simulink model "TP_manual_vrx"  (R2024b)
settings: Solver=FixedStepDiscrete  StartTime=0.0  StopTime=T_end_tp  FixedStep=Ts_tp  RelTol=1e-3
PostLoadFcn:
  | addpath(fileparts(get_param('TP_manual_vrx','FileName')));
InitFcn:
  | TP_manual_init('TP_manual_vrx');
StopFcn:
  | TP_manual_stop('TP_manual_vrx');
values from neighbouring files (symbols this model uses):
  alloc_prm = [half_beam; l_bow; F_max; F_bow_max]    [TP_manual_setup.m]
  D = G.D(1:G.n, :)    [TP_gcs.m]
  d_gps = 0.85    [TP_manual_setup.m]
  lat0_tp = 35.1862095    [TP_manual_setup.m]
  lon0_tp = 128.5665903    [TP_manual_setup.m]
  N_btn = 400    [TP_manual_setup.m]
  S = struct('n', 0)    [TP_gcs.m]    (also in TP_manual_check.m = TP_gcs('result'); TP_manual_stop.m = TP_gcs('result'); TP_mission.m = TP_gcs('result'))
  Ts_tp = 0.05    [TP_manual_setup.m]
  W = 1 - e2*sind(lat0)^2    [TP_gcs.m]    (also in TP_make_video.m = [])
  X_btn = 400    [TP_manual_setup.m]
  Y_btn = 200    [TP_manual_setup.m]
undefined symbols (not defined in the file or in its folder): A, Q
libraries: ros2lib x8
settings Model: Creator=wkyou  LastModifiedBy=wkyou

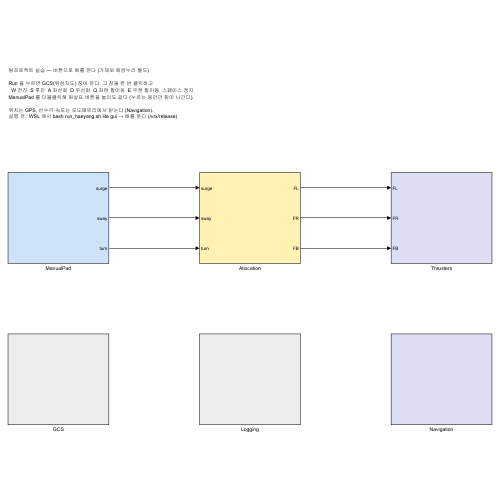
[thumbnail: Simulink's stored preview of the top-level diagram]
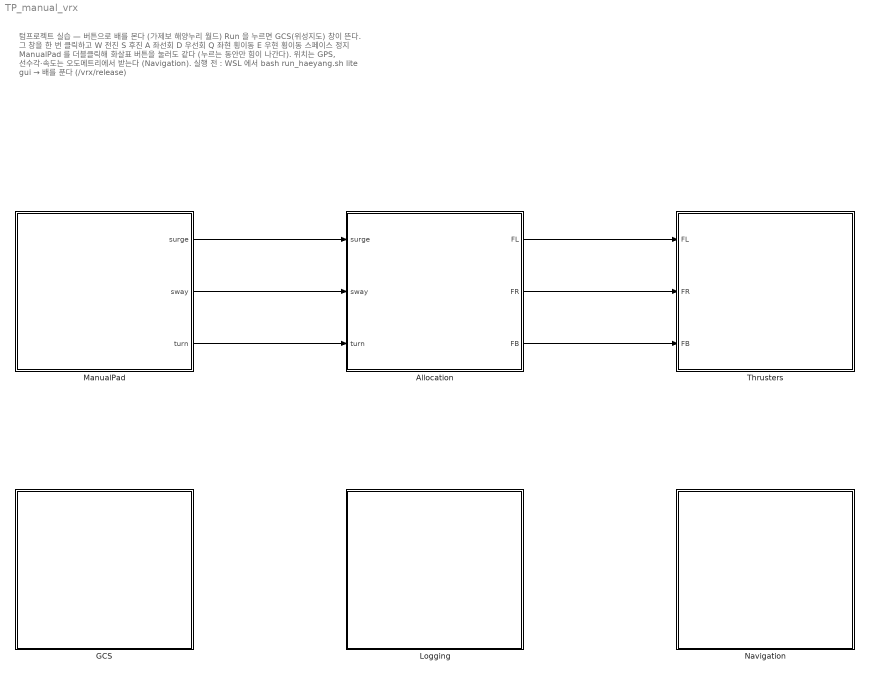
== system TP_manual_vrx ==
  note: 텀프로젝트 실습 — 버튼으로 배를 몬다 (가제보 해양누리 월드)
      |
      | Run 을 누르면 GCS(위성지도) 창이 뜬다. 그 창을 한 번 클릭하고
      |   W 전진  S 후진  A 좌선회  D 우선회  Q 좌현 횡이동  E 우현 횡이동  스페이스 정지
      | ManualPad 를 더블클릭해 화살표 버튼을 눌러도 같다 (누르는 동안만 힘이 나간다).
      |
      | 위치는 GPS, 선수각·속도는 오도메트리에서 받는다 (Navigation).
      | 실행 전 : WSL 에서 bash run_haeyang.sh lite gui → 배를 푼다 (/vrx/release)
  Allocation : Subsystem
  GCS : Subsystem
  Logging : Subsystem
  ManualPad : Subsystem
  Navigation : Subsystem
  Thrusters : Subsystem
  wires:
  ManualPad/1(surge) -> Allocation/1(surge)
  Allocation/1(FL) -> Thrusters/1(FL)
  ManualPad/2(sway) -> Allocation/2(sway)
  Allocation/2(FR) -> Thrusters/2(FR)
  ManualPad/3(turn) -> Allocation/3(turn)
  Allocation/3(FB) -> Thrusters/3(FB)

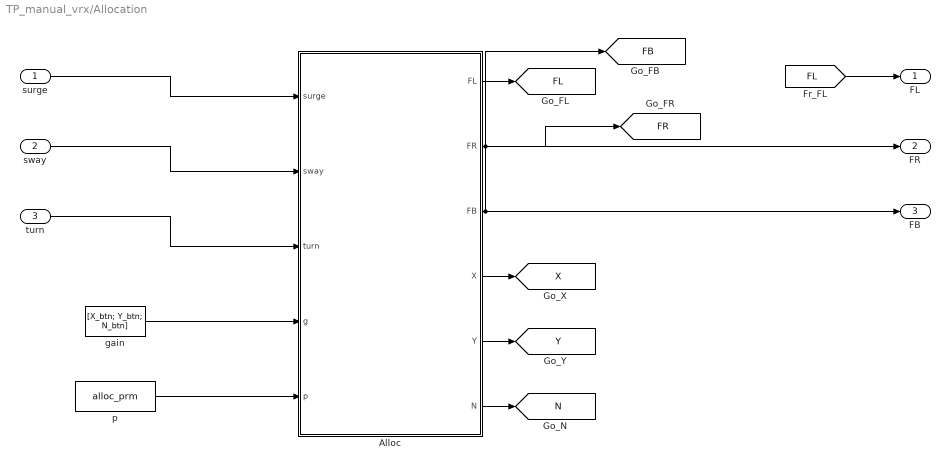
== system TP_manual_vrx/Allocation ==
  surge : Inport
  sway : Inport  Port=2
  turn : Inport  Port=3
  Alloc : MATLAB Function  TreatAsAtomicUnit=on
  gain : Constant  Value=[X_btn; Y_btn; N_btn]
  p : Constant  Value=alloc_prm
  FL : Outport
  FR : Outport  Port=2
  FB : Outport  Port=3
  tag scope: FB=global, FL=global, FR=global, N=global, X=global, Y=global
  wires:
  surge/1 -> Alloc/1(surge)
  sway/1 -> Alloc/2(sway)
  turn/1 -> Alloc/3(turn)
  gain/1 -> Alloc/4(g)
  p/1 -> Alloc/5(p)
  Alloc/2(FR) -> [FR], FR/1
  Alloc/3(FB) -> FB/1, [FB]
  Alloc/1(FL) -> [FL]
  Alloc/6(N) -> [N]
  Alloc/4(X) -> [X]
  Alloc/5(Y) -> [Y]
  [FL] -> FL/1

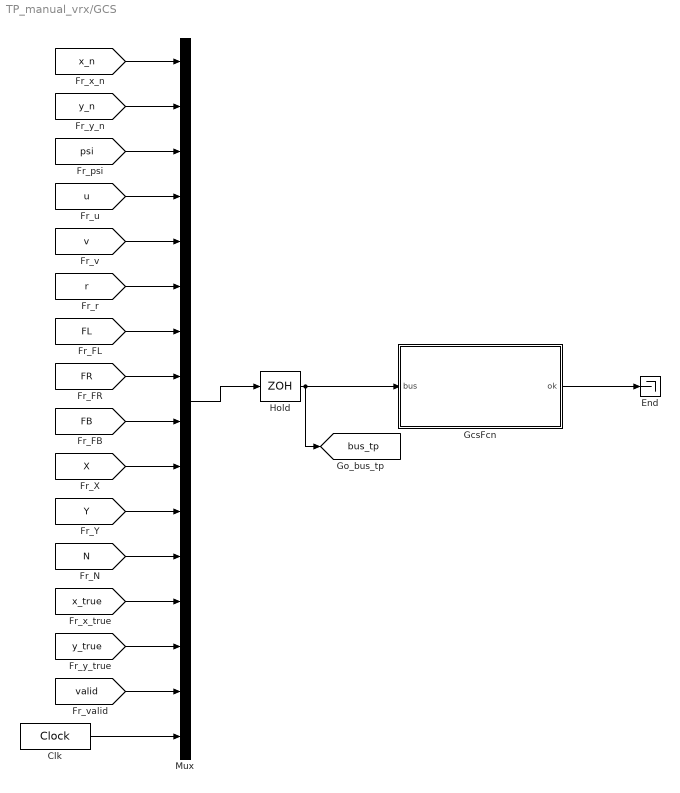
== system TP_manual_vrx/GCS ==
  Clk : DigitalClock  SampleTime=Ts_tp
  End : Terminator
  GcsFcn : MATLAB Function  TreatAsAtomicUnit=on
  Hold : ZeroOrderHold  SampleTime=Ts_tp
  Mux : Mux  Inputs=16
  tag scope: bus_tp=global
  wires:
  Clk/1 -> Mux/16
  Mux/1 -> Hold/1
  Hold/1 -> GcsFcn/1(bus), [bus_tp]
  GcsFcn/1(ok) -> End/1
  [FB] -> Mux/9
  [FL] -> Mux/7
  [FR] -> Mux/8
  [N] -> Mux/12
  [X] -> Mux/10
  [Y] -> Mux/11
  [psi] -> Mux/3
  [r] -> Mux/6
  [u] -> Mux/4
  [v] -> Mux/5
  [valid] -> Mux/15
  [x_n] -> Mux/1
  [x_true] -> Mux/13
  [y_n] -> Mux/2
  [y_true] -> Mux/14

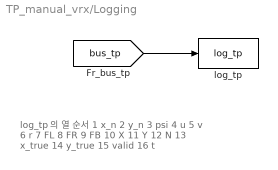
== system TP_manual_vrx/Logging ==
  note: log_tp 의 열 순서
      |  1 x_n   2 y_n   3 psi   4 u   5 v   6 r
      |  7 FL    8 FR    9 FB   10 X  11 Y  12 N
      | 13 x_true  14 y_true  15 valid  16 t
  log_tp : ToWorkspace  VariableName=log_tp  SaveFormat=Timeseries  SampleTime=Ts_tp
  wires:
  [bus_tp] -> log_tp/1

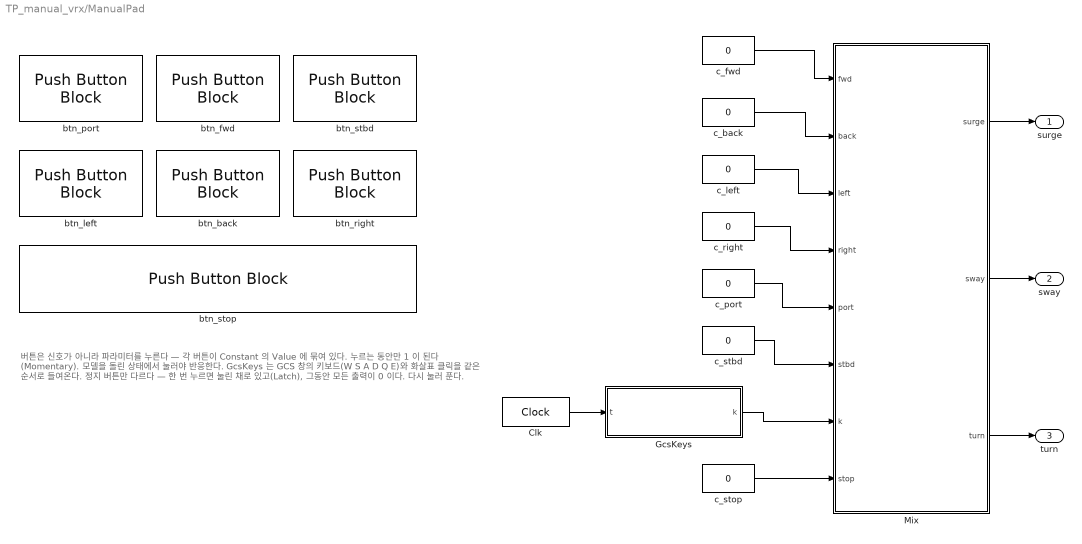
== system TP_manual_vrx/ManualPad ==
  note: 버튼은 신호가 아니라 파라미터를 누른다 — 각 버튼이 Constant 의 Value 에 묶여 있다.
      | 누르는 동안만 1 이 된다 (Momentary). 모델을 돌린 상태에서 눌러야 반응한다.
      | GcsKeys 는 GCS 창의 키보드(W S A D Q E)와 화살표 클릭을 같은 순서로 들여온다.
      | 정지 버튼만 다르다 — 한 번 누르면 눌린 채로 있고(Latch), 그동안 모든 출력이 0 이다. 다시 눌러 푼다.
  Clk : DigitalClock  SampleTime=Ts_tp
  GcsKeys : MATLAB Function  TreatAsAtomicUnit=on
  Mix : MATLAB Function  TreatAsAtomicUnit=on
  btn_back : PushButtonBlock  ButtonText=▼ 후진 (S)
  btn_fwd : PushButtonBlock  ButtonText=▲ 전진 (W)
  btn_left : PushButtonBlock  ButtonText=◀ 좌선회 (A)
  btn_port : PushButtonBlock  ButtonText=⇦ 좌현 횡 (Q)
  btn_right : PushButtonBlock  ButtonText=▶ 우선회 (D)
  btn_stbd : PushButtonBlock  ButtonText=⇨ 우현 횡 (E)
  btn_stop : PushButtonBlock  ButtonText="■ 정지 — 모든 출력 0  (다시 누르면 풀림)"  ButtonType=Latch
  c_back : Constant  Value=0
  c_fwd : Constant  Value=0
  c_left : Constant  Value=0
  c_port : Constant  Value=0
  c_right : Constant  Value=0
  c_stbd : Constant  Value=0
  c_stop : Constant  Value=0
  surge : Outport
  sway : Outport  Port=2
  turn : Outport  Port=3
  wires:
  c_back/1 -> Mix/2(back)
  Clk/1 -> GcsKeys/1(t)
  Mix/3(turn) -> turn/1
  c_fwd/1 -> Mix/1(fwd)
  c_port/1 -> Mix/5(port)
  c_left/1 -> Mix/3(left)
  c_right/1 -> Mix/4(right)
  c_stbd/1 -> Mix/6(stbd)
  c_stop/1 -> Mix/8(stop)
  GcsKeys/1(k) -> Mix/7(k)
  Mix/1(surge) -> surge/1
  Mix/2(sway) -> sway/1

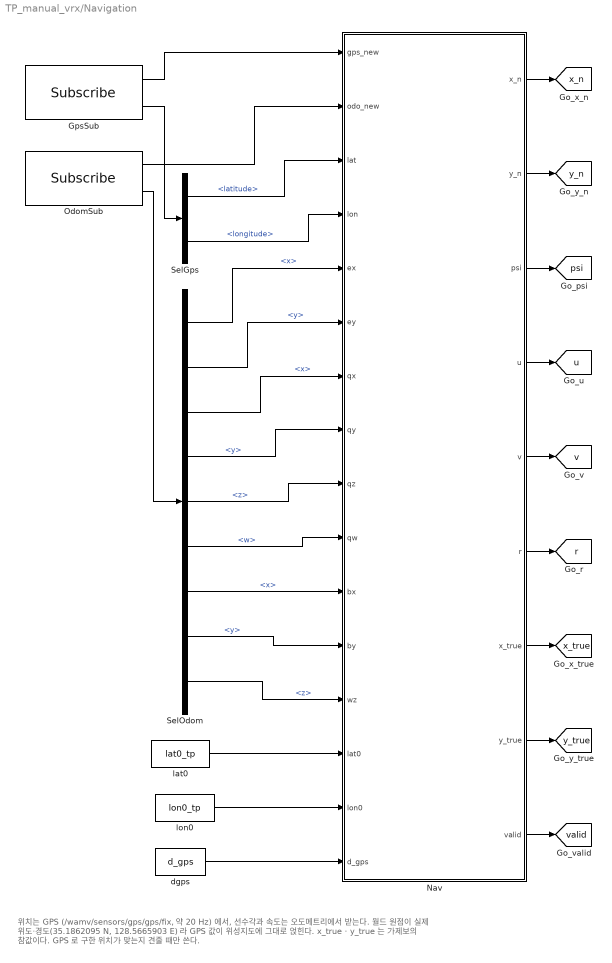
== system TP_manual_vrx/Navigation ==
  note: 위치는 GPS (/wamv/sensors/gps/gps/fix, 약 20 Hz) 에서, 선수각과 속도는 오도메트리에서 받는다.
      | 월드 원점이 실제 위도·경도(35.1862095 N, 128.5665903 E)라 GPS 값이 위성지도에 그대로 얹힌다.
      | x_true · y_true 는 가제보의 참값이다. GPS 로 구한 위치가 맞는지 견줄 때만 쓴다.
  GpsSub : ros2lib/Subscribe  topicSource=Specify your own  topic=/wamv/sensors/gps/gps/fix  messageType=sensor_msgs/NavSatFix  sampleTime=Ts_tp  QOSHistory=Keep last  QOSDepth=1  QOSReliability=Reliable  QOSDurability=Volatile  QOSDeadline=Inf  QOSLifespan=Inf  QOSLiveliness=Automatic  QOSLeaseDuration=Inf  QOSAvoidROSNamespaceConventions=off
  Nav : MATLAB Function  TreatAsAtomicUnit=on
  OdomSub : ros2lib/Subscribe  topicSource=Specify your own  topic=/wamv/sensors/position/ground_truth_odometry  messageType=nav_msgs/Odometry  sampleTime=Ts_tp  QOSHistory=Keep last  QOSDepth=1  QOSReliability=Reliable  QOSDurability=Volatile  QOSDeadline=Inf  QOSLifespan=Inf  QOSLiveliness=Automatic  QOSLeaseDuration=Inf  QOSAvoidROSNamespaceConventions=off
  SelGps : BusSelector  OutputSignals=latitude,longitude
  SelOdom : BusSelector  OutputSignals=pose.pose.position.x,pose.pose.position.y,pose.pose.orientation.x,pose.pose.orientation.y,pose.pose.orientation.z,pose.pose.orientation.w,twist.twist.linear.x,twist.twist.linear.y,twist.twist.angular.z
  dgps : Constant  Value=d_gps
  lat0 : Constant  Value=lat0_tp
  lon0 : Constant  Value=lon0_tp
  tag scope: psi=global, r=global, u=global, v=global, valid=global, x_n=global, x_true=global, y_n=global, y_true=global
  wires:
  OdomSub/2 -> SelOdom/1
  GpsSub/1 -> Nav/1(gps_new)
  SelGps/1 -> Nav/3(lat)  "<latitude>"
  SelOdom/2 -> Nav/6(ey)  "<y>"
  GpsSub/2 -> SelGps/1
  OdomSub/1 -> Nav/2(odo_new)
  SelGps/2 -> Nav/4(lon)  "<longitude>"
  SelOdom/9 -> Nav/13(wz)  "<z>"
  SelOdom/1 -> Nav/5(ex)  "<x>"
  SelOdom/3 -> Nav/7(qx)  "<x>"
  SelOdom/4 -> Nav/8(qy)  "<y>"
  SelOdom/5 -> Nav/9(qz)  "<z>"
  SelOdom/6 -> Nav/10(qw)  "<w>"
  SelOdom/7 -> Nav/11(bx)  "<x>"
  SelOdom/8 -> Nav/12(by)  "<y>"
  lat0/1 -> Nav/14(lat0)
  lon0/1 -> Nav/15(lon0)
  dgps/1 -> Nav/16(d_gps)
  Nav/3(psi) -> [psi]
  Nav/6(r) -> [r]
  Nav/4(u) -> [u]
  Nav/5(v) -> [v]
  Nav/9(valid) -> [valid]
  Nav/1(x_n) -> [x_n]
  Nav/7(x_true) -> [x_true]
  Nav/2(y_n) -> [y_n]
  Nav/8(y_true) -> [y_true]

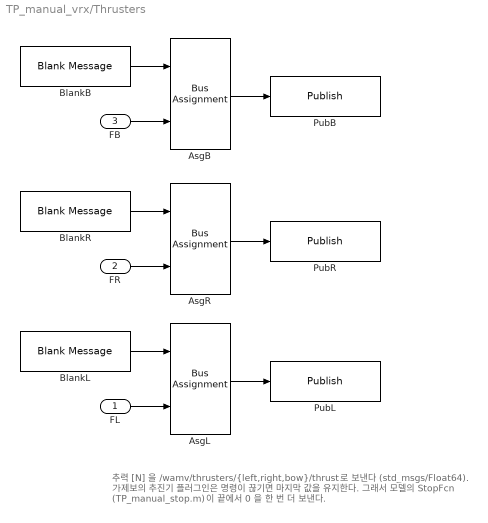
== system TP_manual_vrx/Thrusters ==
  note: 추력 [N] 을 /wamv/thrusters/{left,right,bow}/thrust 로 보낸다 (std_msgs/Float64).
      | 가제보의 추진기 플러그인은 명령이 끊기면 마지막 값을 유지한다.
      | 그래서 모델의 StopFcn (TP_manual_stop.m) 이 끝에서 0 을 한 번 더 보낸다.
  FL : Inport
  FR : Inport  Port=2
  FB : Inport  Port=3
  AsgB : BusAssignment  AssignedSignals=data
  AsgL : BusAssignment  AssignedSignals=data
  AsgR : BusAssignment  AssignedSignals=data
  BlankB : ros2lib/Blank Message  messageClass=Message  entityType=std_msgs/Float64  messageType=std_msgs/Float64  SampleTime=Ts_tp
  BlankL : ros2lib/Blank Message  messageClass=Message  entityType=std_msgs/Float64  messageType=std_msgs/Float64  SampleTime=Ts_tp
  BlankR : ros2lib/Blank Message  messageClass=Message  entityType=std_msgs/Float64  messageType=std_msgs/Float64  SampleTime=Ts_tp
  PubB : ros2lib/Publish  topicSource=Specify your own  topic=/wamv/thrusters/bow/thrust  messageType=std_msgs/Float64  QOSHistory=Keep last  QOSDepth=1  QOSReliability=Reliable  QOSDurability=Volatile  QOSDeadline=Inf  QOSLifespan=Inf  QOSLiveliness=Automatic  QOSLeaseDuration=Inf  QOSAvoidROSNamespaceConventions=off
  PubL : ros2lib/Publish  topicSource=Specify your own  topic=/wamv/thrusters/left/thrust  messageType=std_msgs/Float64  QOSHistory=Keep last  QOSDepth=1  QOSReliability=Reliable  QOSDurability=Volatile  QOSDeadline=Inf  QOSLifespan=Inf  QOSLiveliness=Automatic  QOSLeaseDuration=Inf  QOSAvoidROSNamespaceConventions=off
  PubR : ros2lib/Publish  topicSource=Specify your own  topic=/wamv/thrusters/right/thrust  messageType=std_msgs/Float64  QOSHistory=Keep last  QOSDepth=1  QOSReliability=Reliable  QOSDurability=Volatile  QOSDeadline=Inf  QOSLifespan=Inf  QOSLiveliness=Automatic  QOSLeaseDuration=Inf  QOSAvoidROSNamespaceConventions=off
  wires:
  BlankR/1 -> AsgR/1
  BlankB/1 -> AsgB/1
  FB/1 -> AsgB/2
  FR/1 -> AsgR/2
  BlankL/1 -> AsgL/1
  AsgR/1 -> PubR/1
  AsgB/1 -> PubB/1
  FL/1 -> AsgL/2
  AsgL/1 -> PubL/1

== matlab function TP_manual_vrx/ManualPad/Mix ==
  data: fwd input; surge output; back input; left input; right input; port input; stbd input; k input; stop input; sway output; turn output
function [surge, sway, turn] = Mix(fwd, back, left, right, port, stbd, k, stop)
%#codegen
% 버튼 여섯(이 상자의 Push Button)과 GCS 창의 입력 k 를 합친다.
% 어느 쪽에서 누르든 같다 — 하나라도 눌리면 1.
b = min(1, [fwd; back; left; right; port; stbd] + k);

surge = b(1) - b(2);     % 전진 +1, 후진 -1
sway  = b(6) - b(5);     % 우현 +1, 좌현 -1   (선수추진기가 맡는다)
turn  = b(4) - b(3);     % 우선회 +1 (시계방향), 좌선회 -1

% 정지 버튼이 눌려 있으면 무엇이 눌렸든 0 을 낸다 — 추력 셋이 모두 0 이 된다
if stop > 0.5
    surge = 0;  sway = 0;  turn = 0;
end

== matlab function TP_manual_vrx/ManualPad/GcsKeys ==
  data: t input; k output
function k = GcsKeys(t)
%#codegen
% GCS 창에서 눌린 조종 입력을 읽는다 (TP_gcs_keys.m).
%   k = [전진; 후진; 좌선회; 우선회; 좌현 횡이동; 우현 횡이동],  각 0 또는 1
% 그림 창의 값이라 코드 생성 대상이 아니다. extrinsic 으로 부른다.
coder.extrinsic('TP_gcs_keys');
k = zeros(6, 1);
k = TP_gcs_keys(t);

== matlab function TP_manual_vrx/Allocation/Alloc ==
  data: surge input; FL output; sway input; turn input; g input; p input; FR output; FB output; X output; Y output; N output
function [FL, FR, FB, X, Y, N] = Alloc(surge, sway, turn, g, p)
%#codegen
% 1) 버튼 값(-1 · 0 · +1)에 힘을 곱해 요구 힘·모멘트를 만든다
%      g = [X_btn; Y_btn; N_btn]   버튼 하나가 요구하는 힘 (TP_manual_setup.m)
X = g(1)*surge;          % 전후력 [N]      앞 +
Y = g(2)*sway;           % 횡력 [N]        우현 +
N = g(3)*turn;           % 요 모멘트 [N m] 시계방향 +

% 2) 추력 배분 — 세 추진기로 나눈다 (6주차 W06 의 배분식 그대로)
%      X = FL + FR
%      Y = FB                           횡력은 선수추진기만 낸다
%      N = (FL - FR)*b + l3*FB
%    p = [b; l3; Fmax; Fbmax]
%      b   좌·우 추진기까지의 반폭 [m],  l3  선수추진기의 앞쪽 거리 [m]
%
%    선수추진기가 횡력을 내면 요 모멘트 l3*FB 가 딸려 온다. 그 몫을 좌·우
%    추진기가 되받아 빼야 선수각이 돌지 않는다 — 아래 N - l3*FB 가 그것이다.
b = p(1);  l3 = p(2);  Fmax = p(3);  Fbmax = p(4);
FB = min(max(Y, -Fbmax), Fbmax);
M  = N - l3*FB;          % 포화된 뒤의 FB 로 센다 — 실제로 딸려 온 만큼만 되받는다
FL = X/2 + M/(2*b);
FR = X/2 - M/(2*b);
FL = min(max(FL, -Fmax), Fmax);
FR = min(max(FR, -Fmax), Fmax);

== matlab function TP_manual_vrx/Navigation/Nav ==
  data: gps_new input; x_n output; odo_new input; lat input; lon input; ex input; ey input; qx input; qy input; qz input; qw input; bx input; by input; wz input; lat0 input; lon0 input; d_gps input; y_n output; psi output; u output; v output; r output; x_true output; y_true output; valid output
function [x_n, y_n, psi, u, v, r, x_true, y_true, valid] = Nav(gps_new, odo_new, lat, lon, ex, ey, qx, qy, qz, qw, bx, by, wz, lat0, lon0, d_gps)
%#codegen
% 항법 — 센서 값을 NED 항법량으로 바꾼다.
%   위치 (x_n, y_n)        GPS 위도·경도 → 월드 원점 기준 북·동 [m]
%   선수각 psi · 속도 u v r  오도메트리 (ENU → NED)
%   참값 (x_true, y_true)  오도메트리의 위치. **비교용으로만** 쓴다
%
% 가드 — Subscribe 는 첫 메시지 전에 0 으로 채운 버스를 낸다. 위도 0 · 경도 0 은
% 실제로 있는 곳(기니만)이라 값으로는 가릴 수 없다. IsNew 깃발을 붙잡아 둔다.
persistent seen_gps seen_odo
if isempty(seen_gps), seen_gps = false; seen_odo = false; end
if gps_new, seen_gps = true; end
if odo_new, seen_odo = true; end
valid = double(seen_gps && seen_odo);

% 1) 선수각 — 쿼터니언 → yaw_ENU → psi_NED = pi/2 - yaw_ENU
yaw = atan2(2*(qw*qz + qx*qy), 1 - 2*(qy*qy + qz*qz));
p   = pi/2 - yaw;
psi = atan2(sin(p), cos(p));

% 2) 속도 — y·z 축이 뒤집히므로 부호가 바뀐다
u =  bx;   v = -by;   r = -wz;

% 3) 참값 위치 — ENU 의 y 가 북, x 가 동
x_true = ey;   y_true = ex;

% 4) GPS 위치 — 평면 근사 (A2 부록 예제 5 와 같은 식)
a  = 6378137.0;            % WGS84 장반경 [m]
e2 = 6.69437999014e-3;     % 제1 이심률의 제곱
s2 = sind(lat0)^2;
Rm = a*(1 - e2)/(1 - e2*s2)^1.5;      % 자오선 곡률반경 (남-북)
Rn = a/sqrt(1 - e2*s2);               % 묘유선 곡률반경 (동-서)
xa = (lat - lat0)*pi/180*Rm;                 % 안테나의 북 [m]
ya = (lon - lon0)*pi/180*Rn*cosd(lat0);      % 안테나의 동 [m]

% 5) 안테나 → 선체 중심. 안테나가 중심 뒤 d_gps 에 있으므로 선수 쪽으로 옮긴다
x_n = xa + d_gps*cos(psi);
y_n = ya + d_gps*sin(psi);

if valid < 0.5
    x_n = 0; y_n = 0; psi = 0; u = 0; v = 0; r = 0; x_true = 0; y_true = 0;
end

== matlab function TP_manual_vrx/GCS/GcsFcn ==
  data: bus input; ok output
function ok = GcsFcn(bus)
%#codegen
% GCS 창(위성지도·그래프·조종 버튼)을 부른다 — TP_gcs.m
%   bus = [x_n y_n psi u v r FL FR FB X Y N x_true y_true valid  t]
% 그림은 코드 생성 대상이 아니므로 extrinsic 으로 부른다.
coder.extrinsic('TP_gcs');
ok = 1;
TP_gcs(bus(1:15), bus(16));
